simulink model "labaZB3"  (R2022a)
settings: Solver=VariableStepAuto  StartTime=0.0  StopTime=100  RelTol=1e-3
undefined symbols (not defined in the file): A, B, C, D, K, L, w
settings Model: Creator=User  LastModifiedBy=Roman

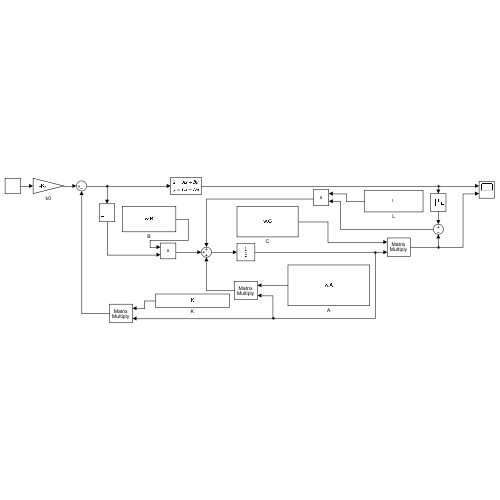
[thumbnail: Simulink's stored preview of the top-level diagram]
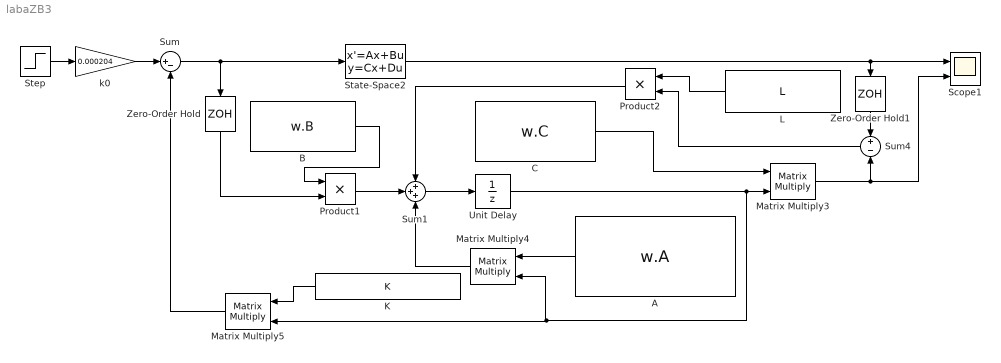
== system labaZB3 ==
  A : Constant  Value=w.A  VectorParams1D=off
  B : Constant  Value=w.B  VectorParams1D=off
  C : Constant  Value=w.C  VectorParams1D=off
  K : Constant  Value=K  VectorParams1D=off
  L : Constant  Value=L  VectorParams1D=off
  Matrix Multiply3 : Product  Multiplication=Matrix(*)
  Matrix Multiply4 : Product  Multiplication=Matrix(*)
  Matrix Multiply5 : Product  Multiplication=Matrix(*)
  Product1 : Product
  Product2 : Product
  Scope1 : Scope  NumInputPorts=2
  State-Space2 : StateSpace  A=A  B=B  C=C  D=D  InitialCondition=[1 1 1]
  Step : Step  Time=0  SampleTime=1
  Sum : Sum  Inputs=|+-
  Sum1 : Sum  Inputs=+++
  Sum4 : Sum  Inputs=+-
  Unit Delay : UnitDelay  SampleTime=10  HasFrameUpgradeWarning=on
  Zero-Order Hold : ZeroOrderHold  SampleTime=10
  Zero-Order Hold1 : ZeroOrderHold  SampleTime=10
  k0 : Gain  Gain=0.000204
  wires:
  Step/1 -> k0/1
  k0/1 -> Sum/1
  Sum/1 -> Zero-Order Hold/1, State-Space2/1
  Zero-Order Hold/1 -> Product1/2
  B/1 -> Product1/1
  Product1/1 -> Sum1/2
  Sum1/1 -> Unit Delay/1
  Unit Delay/1 -> Matrix Multiply5/2, Matrix Multiply4/2, Matrix Multiply3/2
  C/1 -> Matrix Multiply3/1
  Product2/1 -> Sum1/1
  L/1 -> Product2/1
  Sum4/1 -> Product2/2
  Zero-Order Hold1/1 -> Sum4/1
  State-Space2/1 -> Scope1/1, Zero-Order Hold1/1
  A/1 -> Matrix Multiply4/1
  Matrix Multiply4/1 -> Sum1/3
  Matrix Multiply3/1 -> Sum4/2, Scope1/2
  K/1 -> Matrix Multiply5/1
  Matrix Multiply5/1 -> Sum/2
